simulink model "untitled"  (R2025b)
settings: Solver=ode1be  StartTime=0.0  StopTime=15  FixedStep=0.001  RelTol=1e-3
undefined symbols (not defined in the file): DiscIntNeverNeededParam, X, Y, Z
libraries: sm_lib x94, nesl_utility x30, fl_lib x14, ee_lib x5, simulink_extras x4, instrumentseriallib x4, etargetslib x3
(part 4 of 4)

== matlab function untitled/Subsystem1/모터제어기/LeftPid1/MATLAB Left Function ==
  data: PidOutTerm output; User_Vel input; VelErr1 output; Current_Vel input; distance input; PidGain input; AnglePid input; Prev_LPid input; PrevLVelErr1 input; PrevLVelErr2 input; PrevLVelErr3 input; PrevLVelErr4 input; PrevLVelErr input; VelErr2 output; VelErr3 output; VelErr4 output; VelErrSum output
function [PidOutTerm, VelErr1, VelErr2, VelErr3, VelErr4, VelErrSum]= ...
fcn(User_Vel, Current_Vel, distance, PidGain, AnglePid, ...
Prev_LPid, PrevLVelErr1, PrevLVelErr2, PrevLVelErr3, PrevLVelErr4, PrevLVelErr)


Kp = PidGain(1);
Ki = PidGain(2);
Kd = PidGain(3);

VelErr1 = PrevLVelErr1;
VelErr2 = PrevLVelErr2;
VelErr3 = PrevLVelErr3;
VelErr4 = PrevLVelErr4;
VelErrSum = PrevLVelErr;

VelErrSum = VelErrSum - VelErr4;
VelErr4 = VelErr3;
VelErr3 = VelErr2;
VelErr2 = VelErr1;
VelErr1 = -User_Vel*AnglePid;%로봇이 앞으로 기울어졌다 하면
%AnglePid는 - 임. 앞으로 기울면 앞으로 움직여야하기 때문에 Current_Vel이 양수가 됨.
%즉 최종형태는 목표속도(양수)-현재속도(양수)가 되므로 식이 맞음을 알 수 있음.
%pid튜닝 하면서 100을 계속 낮춰보자
%100이 없다라고 가정하자. 로봇이 앞으로 기울면 식의 최종형태는 목표속도(양수)-현재속도(양수)가 되기때문에
%우리가 기대한 식의 결과는 약간 작아진 양수여서(양수끼리 뺄셈) 이 양수가 모터제어로 넘어가서 앞으로 가길 기대함.
%근데 기본적으로 AnglePid와 Current_Vel는 단위가 같지 않기 때문에 Current_Vel가 더 클 때
%식의 결과가 음수가되서 바퀴가 뒤로 굴러서 상황이 심해짐
%만약 이런 상황에서 넘어진다고 하면 AnglePid가 커지기 때문에 다시 식의 결과가 양수가 될 수 있겠지만
%그 양수가 되는 시점이 늦을 수도 있기 때문에 이러한 상황을 방지하고자 Current_Vel에 100을 나눠서
%그런상황이 일어나는걸 방지할 수 있음
%
VelErrSum = VelErrSum + VelErr1;

pid_p = Kp * VelErr1;
pid_i = Ki * VelErrSum;
pid_d = Kd * ((VelErr1 - VelErr4)/0.005+2*(VelErr2-VelErr3)/0.005);

PidOutTerm = 3.5/10*(pid_p + pid_i + pid_d);

V_limit = 20.0; % 정격 전압 설정
if PidOutTerm > V_limit
    PidOutTerm = V_limit;
elseif PidOutTerm < -V_limit
    PidOutTerm = -V_limit;
end

end

== matlab function untitled/Subsystem1/모터제어기/RightPid1/MATLAB Right Function ==
  data: PidOutTerm output; User_Vel input; VelErr1 output; Current_Vel input; distance input; PidGain input; AnglePid input; Prev_RPid input; PrevRVelErr1 input; PrevRVelErr2 input; PrevRVelErr3 input; PrevRVelErr4 input; PrevRVelErr input; VelErr2 output; VelErr3 output; VelErr4 output; VelErrSum output
function [PidOutTerm, VelErr1, VelErr2, VelErr3, VelErr4, VelErrSum]= ...
fcn(User_Vel, Current_Vel, distance, PidGain, AnglePid, ...
Prev_RPid, PrevRVelErr1, PrevRVelErr2, PrevRVelErr3, PrevRVelErr4, PrevRVelErr)


Kp = PidGain(1);
Ki = PidGain(2);
Kd = PidGain(3);

VelErr1 = PrevRVelErr1;
VelErr2 = PrevRVelErr2;
VelErr3 = PrevRVelErr3;
VelErr4 = PrevRVelErr4;
VelErrSum = PrevRVelErr;

VelErrSum = VelErrSum - VelErr4;
VelErr4 = VelErr3;
VelErr3 = VelErr2;
VelErr2 = VelErr1;
VelErr1 = -User_Vel*AnglePid;%로봇이 앞으로 기울어졌다 하면
%AnglePid는 - 임. 앞으로 기울면 앞으로 움직여야하기 때문에 Current_Vel이 양수가 됨.
%즉 최종형태는 목표속도(양수)-현재속도(양수)가 되므로 식이 맞음을 알 수 있음.
%pid튜닝 하면서 100을 계속 낮춰보자
VelErrSum = VelErrSum + VelErr1;

pid_p = Kp * VelErr1;
pid_i = Ki * ((VelErr1 - VelErr4)/0.005+2*(VelErr2-VelErr3)/0.005);
pid_d = Kd * VelErrSum;

PidOutTerm = 3.5/10*(pid_p + pid_i + pid_d);%PidOutTerm은 토크전압Vq임

V_limit = 20.0; % 정격 전압 설정
if PidOutTerm > V_limit
    PidOutTerm = V_limit;
elseif PidOutTerm < -V_limit
    PidOutTerm = -V_limit;
end

end

== matlab function untitled/Subsystem1/물리세계(땅, 로봇)/MATLAB Function2 ==
  data: kp input; wn output; kd input; zeta output; wd output; ts output; N output
function [wn, zeta, wd, ts, N] = fcn(kp, kd)

m = 1;      % 질량 (kg)
g = 9.81;     % 중력가속도 (m/s^2)
L = 0.16;      % 무게중심까지의 거리 (m)
J = m * L^2;  % 관성 모멘트 (kg*m^2)
b = 0.03;     % 시스템 마찰 계수 (실험치)


% 2. 계산 수행
A = (b + kd) / J;
B = (kp - m*g*L) / J;

wn = sqrt(complex(B));%고유진동수
zeta = A / (2 * wn);%감쇠비
wd = wn * sqrt(complex(1 - zeta^2));%감쇠진동수
ts = 4 / (zeta * wn);%전착시간
N = (2 * sqrt(complex(1 - zeta^2))) / (pi * zeta);%진동횟수

end

== matlab function untitled/Subsystem1/모터제어기/LeftPid/MATLAB Left Function ==
  data: PidOutTerm output; User_Vel input; VelErr1 output; Current_Vel input; distance input; PidGain input; AnglePid input; Prev_LPid input; PrevLVelErr1 input; PrevLVelErr2 input; PrevLVelErr3 input; PrevLVelErr4 input; PrevLVelErr input; VelErr2 output; VelErr3 output; VelErr4 output; VelErrSum output
function [PidOutTerm, VelErr1, VelErr2, VelErr3, VelErr4, VelErrSum]= ...
fcn(User_Vel, Current_Vel, distance, PidGain, AnglePid, ...
Prev_LPid, PrevLVelErr1, PrevLVelErr2, PrevLVelErr3, PrevLVelErr4, PrevLVelErr)


Kp = PidGain(1);
Ki = PidGain(2);
Kd = PidGain(3);

VelErr1 = PrevLVelErr1;
VelErr2 = PrevLVelErr2;
VelErr3 = PrevLVelErr3;
VelErr4 = PrevLVelErr4;
VelErrSum = PrevLVelErr;

VelErrSum = VelErrSum - VelErr4;
VelErr4 = VelErr3;
VelErr3 = VelErr2;
VelErr2 = VelErr1;
VelErr1 = -User_Vel*AnglePid;%로봇이 앞으로 기울어졌다 하면
%AnglePid는 - 임. 앞으로 기울면 앞으로 움직여야하기 때문에 Current_Vel이 양수가 됨.
%즉 최종형태는 목표속도(양수)-현재속도(양수)가 되므로 식이 맞음을 알 수 있음.
%pid튜닝 하면서 100을 계속 낮춰보자
%100이 없다라고 가정하자. 로봇이 앞으로 기울면 식의 최종형태는 목표속도(양수)-현재속도(양수)가 되기때문에
%우리가 기대한 식의 결과는 약간 작아진 양수여서(양수끼리 뺄셈) 이 양수가 모터제어로 넘어가서 앞으로 가길 기대함.
%근데 기본적으로 AnglePid와 Current_Vel는 단위가 같지 않기 때문에 Current_Vel가 더 클 때
%식의 결과가 음수가되서 바퀴가 뒤로 굴러서 상황이 심해짐
%만약 이런 상황에서 넘어진다고 하면 AnglePid가 커지기 때문에 다시 식의 결과가 양수가 될 수 있겠지만
%그 양수가 되는 시점이 늦을 수도 있기 때문에 이러한 상황을 방지하고자 Current_Vel에 100을 나눠서
%그런상황이 일어나는걸 방지할 수 있음
%
VelErrSum = VelErrSum + VelErr1;

pid_p = Kp * VelErr1;
pid_i = Ki * VelErrSum;
pid_d = Kd * ((VelErr1 - VelErr4)/0.005+2*(VelErr2-VelErr3)/0.005);

PidOutTerm = 3.5/10*(pid_p + pid_i + pid_d);

V_limit = 20.0; % 정격 전압 설정
if PidOutTerm > V_limit
    PidOutTerm = V_limit;
elseif PidOutTerm < -V_limit
    PidOutTerm = -V_limit;
end

end

== matlab function untitled/Subsystem1/각도제어기/PitchPIDout/MATLAB Function ==
  data: PitchOutTerm output; PitchErr1 output; PitchErr2 output; PitchErr3 output; PitchErr4 output; PitchErrSum output; Userpitch input; Pid_Gain input; Pitch input; VelSum input; PrevPidOut input; PrevPitchErr1 input; PrevPitchErr2 input; PrevPitchErr3 input; PrevPitchErr4 input; PrevPitchErrSum input
function [PitchOutTerm, PitchErr1, PitchErr2, PitchErr3, PitchErr4, PitchErrSum] = ... %출력
fcn(Userpitch, Pid_Gain, Pitch, VelSum, PrevPidOut, PrevPitchErr1,...                  %입력
PrevPitchErr2, PrevPitchErr3, PrevPitchErr4, PrevPitchErrSum)

kp = Pid_Gain(1);
ki = Pid_Gain(2);
kd = Pid_Gain(3);

PitchErrSum = PrevPitchErrSum;
PitchErr4 = PrevPitchErr4;
PitchErr3 = PrevPitchErr3;
PitchErr2 = PrevPitchErr2;
PitchErr1 = PrevPitchErr1;

%next_pitch = -(VelSum/90) + Userpitch;

%if(next_pitch > 30)
%    next_pitch = 30;
%elseif(next_pitch < -30)
%    next_pitch = -30;
%end

%PitchErrSum = PitchErrSum - PitchErr4;
PitchErr4 = PitchErr3;%이이이전오차
PitchErr3 = PitchErr2;%이이전오차
PitchErr2 = PitchErr1;%이전오차
PitchErr1 = Userpitch - Pitch;%현재오차
PitchErrSum = PitchErrSum + PitchErr1;

pid_p = kp*PitchErr1;%비례
pid_i = ki*(PitchErrSum);%적분
pid_d = kd*((PitchErr1 - PitchErr4)/0.005 + 2*(PitchErr2 - PitchErr3)/0.005);%미분

PitchOutTerm = pid_p + pid_i + pid_d; %단위: rad(라디안은 무차원임)
%PitchOutTerm = PrevPidOut + pid_p + pid_i + pid_d;
end

== matlab function untitled/Subsystem1/모터제어기/RightPid/MATLAB Right Function ==
  data: PidOutTerm output; User_Vel input; VelErr1 output; Current_Vel input; distance input; PidGain input; AnglePid input; Prev_RPid input; PrevRVelErr1 input; PrevRVelErr2 input; PrevRVelErr3 input; PrevRVelErr4 input; PrevRVelErr input; VelErr2 output; VelErr3 output; VelErr4 output; VelErrSum output
function [PidOutTerm, VelErr1, VelErr2, VelErr3, VelErr4, VelErrSum]= ...
fcn(User_Vel, Current_Vel, distance, PidGain, AnglePid, ...
Prev_RPid, PrevRVelErr1, PrevRVelErr2, PrevRVelErr3, PrevRVelErr4, PrevRVelErr)


Kp = PidGain(1);
Ki = PidGain(2);
Kd = PidGain(3);

VelErr1 = PrevRVelErr1;
VelErr2 = PrevRVelErr2;
VelErr3 = PrevRVelErr3;
VelErr4 = PrevRVelErr4;
VelErrSum = PrevRVelErr;

VelErrSum = VelErrSum - VelErr4;
VelErr4 = VelErr3;
VelErr3 = VelErr2;
VelErr2 = VelErr1;
VelErr1 = -User_Vel*AnglePid;%로봇이 앞으로 기울어졌다 하면
%AnglePid는 - 임. 앞으로 기울면 앞으로 움직여야하기 때문에 Current_Vel이 양수가 됨.
%즉 최종형태는 목표속도(양수)-현재속도(양수)가 되므로 식이 맞음을 알 수 있음.
%pid튜닝 하면서 100을 계속 낮춰보자
VelErrSum = VelErrSum + VelErr1;

pid_p = Kp * VelErr1;
pid_i = Ki * ((VelErr1 - VelErr4)/0.005+2*(VelErr2-VelErr3)/0.005);
pid_d = Kd * VelErrSum;

PidOutTerm = 3.5/10*(pid_p + pid_i + pid_d);%PidOutTerm은 토크전압Vq임

V_limit = 20.0; % 정격 전압 설정
if PidOutTerm > V_limit
    PidOutTerm = V_limit;
elseif PidOutTerm < -V_limit
    PidOutTerm = -V_limit;
end

end

== matlab function untitled/Subsystem1/각도제어기/YawPIDout/MATLAB Function ==
  data: PitchOutTerm output; YawErr1 output; YawErr2 output; YawErr3 output; YawErr4 output; YawErrSum output; UserYaw input; Pid_Gain input; Yaw input; PrevPidOut input; PrevYawErr1 input; PrevYawErr2 input; PrevYawErr3 input; PrevYawErr4 input; PrevYawErrSum input
function [PitchOutTerm, YawErr1, YawErr2, YawErr3, YawErr4, YawErrSum] = ... %출력
fcn(UserYaw, Pid_Gain, Yaw, PrevPidOut, PrevYawErr1,...                  %입력
PrevYawErr2, PrevYawErr3, PrevYawErr4, PrevYawErrSum)

kp = Pid_Gain(1);
ki = Pid_Gain(2);
kd = Pid_Gain(3);

YawErrSum = PrevYawErrSum;
YawErr4 = PrevYawErr4;
YawErr3 = PrevYawErr3;
YawErr2 = PrevYawErr2;
YawErr1 = PrevYawErr1;

%if(next_pitch > 30)
%    next_pitch = 30;
%elseif(next_pitch < -30)
%    next_pitch = -30;
%end

YawErrSum = YawErrSum - YawErr4;
YawErr4 = YawErr3;
YawErr3 = YawErr2;
YawErr2 = YawErr1;
YawErr1 = UserYaw - Yaw;
YawErrSum = YawErrSum + YawErr1;

pid_p = kp*YawErr1;
pid_i = ki*YawErrSum;
pid_d = kd*((YawErr1 - YawErr4)/0.005 + 2*(YawErr2 - YawErr3)/0.005);

PitchOutTerm = pid_p + pid_i + pid_d; %단위: rad(라디안은 무차원임)
%PitchOutTerm = PrevPidOut + pid_p + pid_i + pid_d;
end
